simulink model "Universal_ELC_for_MicroHydoPlant"  (R2025a)
settings: Solver=ode45  StartTime=0.0  StopTime=2  RelTol=1e-3
undefined symbols (not defined in the file): R_user
libraries: spsCurrentMeasurementLib x13, spsSeriesRLCBranchLib x9, spsMosfetLib x7, spsVoltageMeasurementLib x5, spsUniversalBridgeLib x3, spsPower3phInstantaneousLib x3, spsControlledVoltageSourceLib x3, spsThreePhaseSeriesRLCBranchLib x2, slpidlib x2, spsTHDLib x2, spsRMSLib x1, spsGroundLib x1
settings Model: Creator=Niranjan  LastModifiedBy=SimuVerity Contributors
settings SolverCC: AlgebraicLoopSolver=TrustRegion
settings DataIOCC: SaveFormat=StructureWithTime  ReturnWorkspaceOutputs=off
settings OptimizationCC: LifeSpan=inf
settings DebuggingCC: UnconnectedInputMsg=warning  UnconnectedOutputMsg=warning  UnconnectedLineMsg=warning  SFExecutionAtInitializationDiag=none  ArithmeticOperatorsInVariantConditions=warning
settings HardwareCC: ProdBitPerSizeT=32.0  ProdBitPerPtrDiffT=32.0  ProdWordSize=32.0  ProdHWDeviceType=Specified
settings ModelReferenceCC: EnableRefExpFcnMdlSchedulingChecks=on
settings SFSimCC: SimUseLocalCustomCode=off  CustomCodeUndefinedFunction=UseInterfaceOnly
settings RTWCC: RTWUseLocalCustomCode=off  GPUComputeCapability=3.5
settings CodeAppCC: StateflowObjectComments=on
settings SimscapeCC: SimscapeNormalizeSystem=off

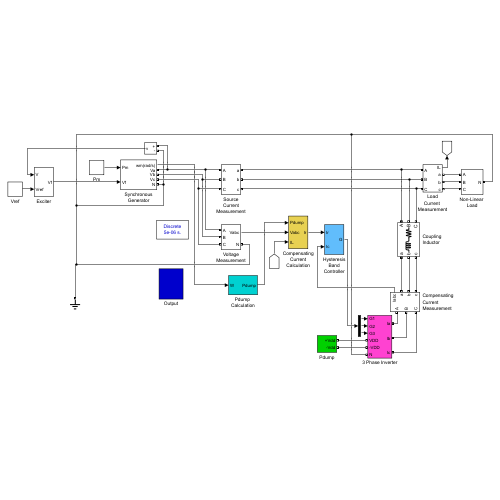
[thumbnail: Simulink's stored preview of the top-level diagram]
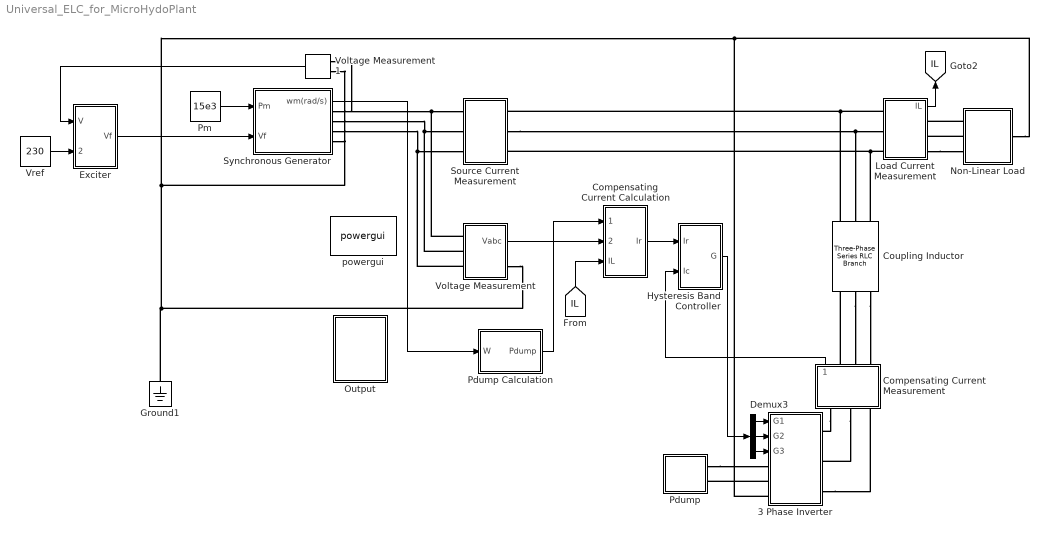
== system Universal_ELC_for_MicroHydoPlant ==
  3 Phase Inverter : Subsystem
  Compensating Current Calculation : Subsystem
  Compensating Current Measurement : Subsystem
  Coupling Inductor : spsThreePhaseSeriesRLCBranchLib/Three-Phase Series RLC Branch  LConnTagsString=A|B|C  RConnTagsString=A|B|C  BranchType=RL  Resistance=0.5  Inductance=0.015  Capacitance=1e-6  Measurements=None
  Demux3 : Demux  Outputs=3
  Exciter : Subsystem
  Ground1 : spsGroundLib/Ground  LConnTagsString=a
  Hysteresis Band Controller : Subsystem
  Load Current Measurement : Subsystem
  "Non-Linear Load " : Subsystem
  Output : Subsystem
  Pdump : Subsystem
  Pdump Calculation : Subsystem
  Pm : Constant  Value=15e3
  Source Current Measurement : Subsystem
  Synchronous Generator : Subsystem
  Voltage Measurement : Subsystem
  Voltage Measurement1 : spsVoltageMeasurementLib/Voltage Measurement  PhasorSimulation=off  OutputType=Complex  PSBequivalent=0
  Vref : Constant  Value=230
  powergui : spspowerguiLib/powergui  Priority=1  SimulationMode=Discrete  SampleTime=5e-6  frequency=60  Iterations=50  frequencyindice=0  Pbase=100e6  ErrMax=1e-4  UnitsV=kV  UnitsW=MW  buscounter=0  FunctionMessages=off  echomessages=off  EnableUseOfTLC=off  CurrentSourceSwitches=off  DisableSnubberDevices=off  DisableRonSwitches=off  DisableVfSwitches=off  DisplayEquations=off  AutomaticDiscreteSolvers=off  SolverType=Backward Euler  Interpol=off  ExternalGateDelay=off  methode=off  Ts=0  x0status=blocks  SPID=off  SwTol=0  HookPort=off  NonlinearTolerance=1e-4  nMaxIteration=100  ContinueOnMaxIteration=off  RestoreLinks=warning  ResistiveCurrentMeasurement=off  Frange=[0:2:500]  Ylog=off  Xlog=on  ShowGrid=off  save=off  variable=ZData  structure=0  ZoomFFT=off  StartTime=0.0  cycles=1  DisplayStyle=1  fundamental=60  FreqAxis=off  MaxFrequency=1000  frequencyindicesteady=1  RmsSteady=1  display=off
  tag scope: IL=global
  wires:
  Demux3/1 -> 3 Phase Inverter/1(G1)
  Demux3/2 -> 3 Phase Inverter/2(G2)
  Demux3/3 -> 3 Phase Inverter/3(G3)
  Hysteresis Band Controller/1(G) -> Demux3/1
  Compensating Current Measurement/1(Iabc) -> Hysteresis Band Controller/2(Ic)
  Compensating Current Calculation/1(Ir) -> Hysteresis Band Controller/1(Ir)
  Pdump Calculation/1(Pdump) -> Compensating Current Calculation/1(Pdump)
  Voltage Measurement/1(Vabc) -> Compensating Current Calculation/2(Vabc)
  Load Current Measurement/1(IL) -> [IL]
  [IL] -> Compensating Current Calculation/3(IL)
  Pm/1 -> Synchronous Generator/1(Pm)
  Synchronous Generator/1(wm(rad/s)) -> Pdump Calculation/1(W)
  Voltage Measurement1/1 -> Exciter/1(V)
  Vref/1 -> Exciter/2(Vref)
  Exciter/1(Vf) -> Synchronous Generator/2(Vf)
  connections:
  Compensating Current Measurement/LConn1 -- 3 Phase Inverter/RConn1
  Voltage Measurement/LConn1 -- Voltage Measurement1/LConn1 -- Synchronous Generator/RConn1 -- Source Current Measurement/LConn1
  3 Phase Inverter/RConn3 -- Compensating Current Measurement/LConn3
  Compensating Current Measurement/LConn2 -- 3 Phase Inverter/RConn2
  Compensating Current Measurement/RConn1 -- Coupling Inductor/RConn1
  Coupling Inductor/RConn2 -- Compensating Current Measurement/RConn2
  "Non-Linear Load "/LConn1 -- Load Current Measurement/RConn1
  Coupling Inductor/RConn3 -- Compensating Current Measurement/RConn3
  Load Current Measurement/RConn3 -- "Non-Linear Load "/LConn3
  Voltage Measurement/LConn2 -- Synchronous Generator/RConn2 -- Source Current Measurement/LConn2
  Pdump/RConn1 -- 3 Phase Inverter/LConn1
  3 Phase Inverter/LConn2 -- Pdump/RConn2
  Load Current Measurement/LConn1 -- Coupling Inductor/LConn1 -- Source Current Measurement/RConn1
  Load Current Measurement/LConn3 -- Coupling Inductor/LConn3 -- Source Current Measurement/RConn3
  Voltage Measurement/LConn3 -- Synchronous Generator/RConn3 -- Source Current Measurement/LConn3
  Voltage Measurement/RConn1 -- Ground1/LConn1 -- Voltage Measurement1/LConn2 -- Synchronous Generator/RConn4 -- "Non-Linear Load "/RConn1 -- 3 Phase Inverter/LConn3
  Source Current Measurement/RConn2 -- Coupling Inductor/LConn2 -- Load Current Measurement/LConn2
  "Non-Linear Load "/LConn2 -- Load Current Measurement/RConn2

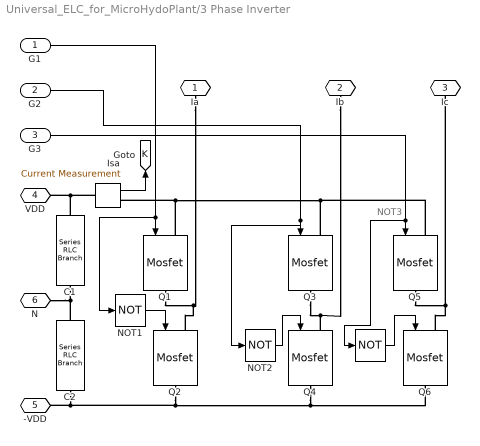
== system Universal_ELC_for_MicroHydoPlant/3 Phase Inverter ==
  note: NOT3
  G1 : Inport
  G2 : Inport  Port=2
  G3 : Inport  Port=3
  " " : Logic  Operator=NOT  AllPortsSameDT=off  OutDataTypeStr=boolean
  C1 : spsSeriesRLCBranchLib/Series RLC Branch  LConnTagsString=__new0  RConnTagsString=__new0  BranchType=C  Resistance=1  Inductance=1e-3  SetiL0=off  InitialCurrent=0  Capacitance=4700e-6  Setx0=on  InitialVoltage=500  Measurements=None
  C2 : spsSeriesRLCBranchLib/Series RLC Branch  LConnTagsString=__new0  RConnTagsString=__new0  BranchType=C  Resistance=1  Inductance=1e-3  SetiL0=off  InitialCurrent=0  Capacitance=4700e-6  Setx0=on  InitialVoltage=500  Measurements=None
  Isa : spsCurrentMeasurementLib/Current Measurement  PhasorSimulation=off  OutputType=Complex  PSBequivalent=0
  NOT1 : Logic  Operator=NOT  AllPortsSameDT=off  OutDataTypeStr=boolean
  NOT2 : Logic  Operator=NOT  AllPortsSameDT=off  OutDataTypeStr=boolean
  Q{1..6} (6 alike) : spsMosfetLib/Mosfet  Ron=0.01  Lon=0  Rd=0.01  Vfd=0  IC=0  Rs=1e10  Cs=inf  Measurements=off
  Ia : PMIOPort  Side=Right
  Ib : PMIOPort  Port=2  Side=Right
  Ic : PMIOPort  Port=3  Side=Right
  VDD : PMIOPort  Port=4  Side=Left
  -VDD : PMIOPort  Port=5  Side=Left
  N : PMIOPort  Port=6  Side=Left
  tag scope: K=global
  wires:
  NOT1/1 -> Q2/1
  NOT2/1 -> Q4/1
  " "/1 -> Q6/1
  G1/1 -> NOT1/1, Q1/1
  G2/1 -> Q3/1, NOT2/1
  G3/1 -> Q5/1, " "/1
  Isa/1 -> [K]
  connections:
  Q1/RConn1 -- Ia/RConn1 -- Q2/LConn1
  Isa/LConn1 -- VDD/RConn1 -- C1/LConn1
  Q3/RConn1 -- Ib/RConn1 -- Q4/LConn1
  Q2/RConn1 -- C2/RConn1 -- -VDD/RConn1 -- Q4/RConn1 -- Q6/RConn1
  Q6/LConn1 -- Ic/RConn1 -- Q5/RConn1
  Q1/LConn1 -- Isa/RConn1 -- Q5/LConn1 -- Q3/LConn1
  C2/LConn1 -- C1/RConn1 -- N/RConn1

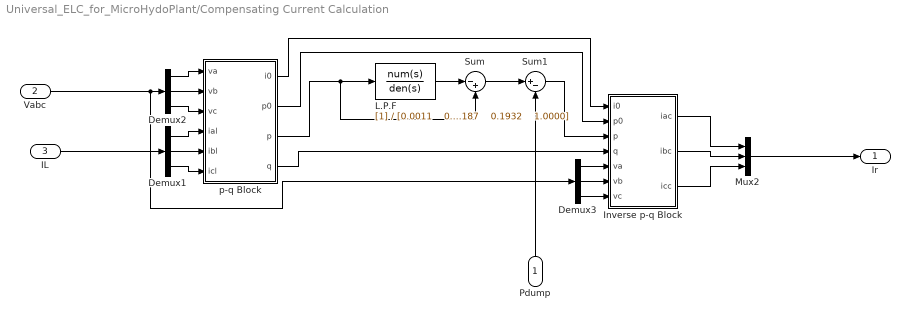
== system Universal_ELC_for_MicroHydoPlant/Compensating Current Calculation ==
  Pdump : Inport
  Vabc : Inport  Port=2
  IL : Inport  Port=3
  Demux1 : Demux  Outputs=3
  Demux2 : Demux  Outputs=3
  Demux3 : Demux  Outputs=3
  Inverse p-q Block : MATLAB Function  TreatAsAtomicUnit=on
  L.P.F : TransferFcn  Denominator="[0.0011    0.0187    0.1932    1.0000]"
  Mux2 : Mux  Inputs=3
  Sum : Sum  Inputs=|-+
  Sum1 : Sum  Inputs=|+-
  p-q Block : MATLAB Function  TreatAsAtomicUnit=on
  Ir : Outport
  wires:
  Inverse p-q Block/3(icc) -> Mux2/3
  IL/1 -> Demux1/1
  Demux1/2 -> p-q Block/5(ibl)
  Mux2/1 -> Ir/1
  Inverse p-q Block/1(iac) -> Mux2/1
  Demux1/1 -> p-q Block/4(ial)
  Inverse p-q Block/2(ibc) -> Mux2/2
  p-q Block/1(i0) -> Inverse p-q Block/1(i0)
  p-q Block/3(p) -> L.P.F/1, Sum/2
  Pdump/1 -> Sum1/2
  L.P.F/1 -> Sum/1
  Sum/1 -> Sum1/1
  Sum1/1 -> Inverse p-q Block/3(p)
  p-q Block/4(q) -> Inverse p-q Block/4(q)
  Demux1/3 -> p-q Block/6(icl)
  p-q Block/2(p0) -> Inverse p-q Block/2(p0)
  Demux2/3 -> p-q Block/3(vc)
  Demux2/2 -> p-q Block/2(vb)
  Demux2/1 -> p-q Block/1(va)
  Vabc/1 -> Demux3/1, Demux2/1
  Demux3/1 -> Inverse p-q Block/5(va)
  Demux3/2 -> Inverse p-q Block/6(vb)
  Demux3/3 -> Inverse p-q Block/7(vc)

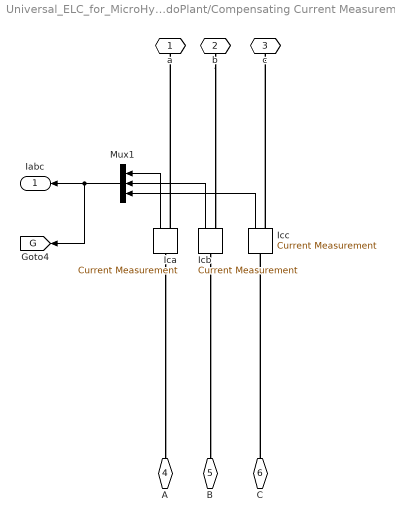
== system Universal_ELC_for_MicroHydoPlant/Compensating Current Measurement ==
  Ica : spsCurrentMeasurementLib/Current Measurement  PhasorSimulation=off  OutputType=Complex  PSBequivalent=0
  Icb : spsCurrentMeasurementLib/Current Measurement  PhasorSimulation=off  OutputType=Complex  PSBequivalent=0
  Icc : spsCurrentMeasurementLib/Current Measurement  PhasorSimulation=off  OutputType=Complex  PSBequivalent=0
  Mux1 : Mux  Inputs=3
  a : PMIOPort  Side=Right
  b : PMIOPort  Port=2  Side=Right
  c : PMIOPort  Port=3  Side=Right
  A : PMIOPort  Port=4  Side=Left
  B : PMIOPort  Port=5  Side=Left
  C : PMIOPort  Port=6  Side=Left
  Iabc : Outport
  tag scope: G=global
  wires:
  Mux1/1 -> [G], Iabc/1
  Ica/1 -> Mux1/1
  Icc/1 -> Mux1/3
  Icb/1 -> Mux1/2
  connections:
  b/RConn1 -- Icb/RConn1
  Ica/RConn1 -- a/RConn1
  Icc/RConn1 -- c/RConn1
  C/RConn1 -- Icc/LConn1
  Ica/LConn1 -- A/RConn1
  Icb/LConn1 -- B/RConn1

== system Universal_ELC_for_MicroHydoPlant/Exciter ==
  V : Inport
  Vref : Inport  Port=2
  PI Controller : slpidlib/PID Controller  Controller=PI  Form=Parallel  TimeDomain=Continuous-time  UseExternalTs=off  SampleTime=-1  IntegratorMethod=Forward Euler  FilterMethod=Forward Euler  ControllerParametersSource=internal  P=8  I=6  UseKiTs=off  D=0  UseExternalDerivativeSource=off  N=100  UseFilter=on  TunerSelectOption=Transfer Function Based (PID Tuner App)  InitialConditionSource=internal  InitialConditionForIntegrator=0  InitialConditionForFilter=0  DifferentiatorICPrevScaledInput=0  ExternalReset=none  TrackingMode=off  Kt=1  LimitOutput=off  SatLimitsSource=internal  UpperSaturationLimit=inf  LowerSaturationLimit=-inf  LinearizeAsGain=on  AntiWindupMode=none  Kb=1  LimitIntegrator=off  UpperIntegratorSaturationLimit=inf  LowerIntegratorSaturationLimit=-inf  POutMin=[]  POutMax=[]  IOutMin=[]  IOutMax=[]  DOutMin=[]  DOutMax=[]  NOutMin=[]  NOutMax=[]  SumOutMin=[]  SumOutMax=[]  SaturationOutMin=[]  SaturationOutMax=[]  PParamMin=[]  PParamMax=[]  IParamMin=[]  IParamMax=[]  DParamMin=[]  DParamMax=[]  NParamMin=[]  NParamMax=[]  KbParamMin=[]  KbParamMax=[]  KtParamMin=[]  KtParamMax=[]  KbOutMin=[]  KbOutMax=[]  KtOutMin=[]  KtOutMax=[]  IntegratorOutMin=[]  IntegratorOutMax=[]  FilterOutMin=[]  FilterOutMax=[]  SumI1OutMin=[]  SumI1OutMax=[]  SumI2OutMin=[]  SumI2OutMax=[]  SumI3OutMin=[]  SumI3OutMax=[]  SumI4OutMin=[]  SumI4OutMax=[]  SumDOutMin=[]  SumDOutMax=[]  DifferentiatorOutMin=[]  DifferentiatorOutMax=[]  FilterDiffOutCoefMin=[]  FilterDiffOutCoefMax=[]  ReciprocalOutMin=[]  ReciprocalOutMax=[]  SumDenOutMin=[]  SumDenOutMax=[]  SumNumOutMin=[]  SumNumOutMax=[]  DivideOutMin=[]  DivideOutMax=[]  UdiffTsProdOutMin=[]  UdiffTsProdOutMax=[]  NTsProdOutMin=[]  NTsProdOutMax=[]  UintegralTsProdOutMin=[]  UintegralTsProdOutMax=[]  UngainTsProdOutMin=[]  UngainTsProdOutMax=[]  ClampingZeroOutDataTypeStr=Inherit: Inherit via back propagation  ClampingZeroOutMin=[]  ClampingZeroOutMax=[]  FilterDenConstantOutDataTypeStr=Inherit: Inherit via back propagation  FilterDenConstantOutMin=[]  FilterDenConstantOutMax=[]  PCopyOutDataTypeStr=Inherit: Inherit via back propagation  PCopyOutMin=[]  PCopyOutMax=[]  NCopyOutDataTypeStr=Inherit: Inherit via back propagation  NCopyOutMin=[]  NCopyOutMax=[]  IntegratorContinuousStateAttributes=''  IntegratorStateMustResolveToSignalObject=off  IntegratorRTWStateStorageClass=Auto  FilterContinuousStateAttributes=''  FilterStateMustResolveToSignalObject=off  FilterRTWStateStorageClass=Auto  ParallelPVariant=InternalParameters  IdealPVariant=Disabled  IVariant=InternalParameters  DVariant=Disabled  IntegratorVariant=Continuous  SatVariant=Disabled  AWVariant=Passthrough  PCopyVariant=Disabled  TRVariant=Disabled  FdbkBlocksVariant=Forward  IdealPFdbkVariant=Disabled  SatFdbkVariant=Disabled  DerivativeFilterVariant=Disabled  NVariant=Disabled  NCopyVariant=Disabled_SignalSpec  FilterICVariant=Disabled  IntegratorICVariant=InternalICs  ExternalResetVariant=Disabled  TRSumVariant=Passthrough  SumFdbkVariant=Disabled  SumVariant=Sum_PI  TsampFilterVariant=InternalTs  TsampNgainVariant=Passthrough  TsampIntegralVariant=Disabled_SignalSpec  ExternalSaturationOutDataTypeStr=Inherit: Same as second input  DerivativeSourceVariant=Disabled  PreIntVariant=InternalPreInt
  RMS : spsRMSLib/RMS  TrueRMS=on  Freq=50  RMSInit=120  Ts=0
  Sum : Sum  Inputs=-+|
  Vf : Outport
  wires:
  V/1 -> RMS/1
  PI Controller/1 -> Vf/1
  Sum/1 -> PI Controller/1
  RMS/1 -> Sum/1
  Vref/1 -> Sum/2

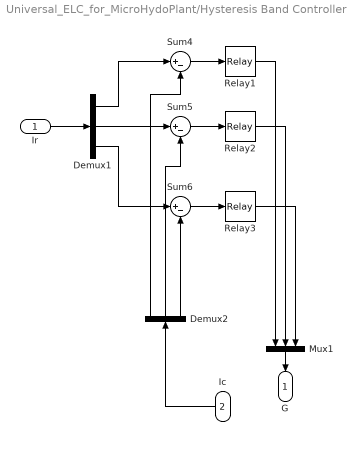
== system Universal_ELC_for_MicroHydoPlant/Hysteresis Band Controller ==
  Ir : Inport
  Ic : Inport  Port=2
  Demux1 : Demux  Outputs=3
  Demux2 : Demux  Outputs=3
  Mux1 : Mux  Inputs=3
  Relay1 : Relay  OnSwitchValue=0.1  OffSwitchValue=-0.2  ZeroCross=off
  Relay2 : Relay  OnSwitchValue=0.2  OffSwitchValue=-0.2  ZeroCross=off
  Relay3 : Relay  OnSwitchValue=0.2  OffSwitchValue=-0.2  ZeroCross=off
  Sum4 : Sum  Inputs=|+-
  Sum5 : Sum  Inputs=|+-
  Sum6 : Sum  Inputs=|+-
  G : Outport
  wires:
  Relay3/1 -> Mux1/3
  Relay1/1 -> Mux1/1
  Relay2/1 -> Mux1/2
  Demux2/2 -> Sum5/2
  Demux1/2 -> Sum5/1
  Sum6/1 -> Relay3/1
  Demux1/1 -> Sum4/1
  Demux1/3 -> Sum6/1
  Demux2/3 -> Sum6/2
  Sum5/1 -> Relay2/1
  Demux2/1 -> Sum4/2
  Sum4/1 -> Relay1/1
  Mux1/1 -> G/1
  Ir/1 -> Demux1/1
  Ic/1 -> Demux2/1

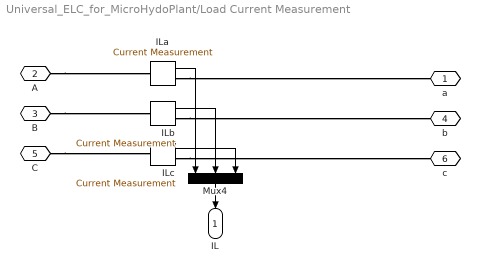
== system Universal_ELC_for_MicroHydoPlant/Load Current Measurement ==
  ILa : spsCurrentMeasurementLib/Current Measurement  PhasorSimulation=off  OutputType=Complex  PSBequivalent=0
  ILb : spsCurrentMeasurementLib/Current Measurement  PhasorSimulation=off  OutputType=Complex  PSBequivalent=0
  ILc : spsCurrentMeasurementLib/Current Measurement  PhasorSimulation=off  OutputType=Complex  PSBequivalent=0
  Mux4 : Mux  Inputs=3
  a : PMIOPort  Side=Right
  A : PMIOPort  Port=2  Side=Left
  B : PMIOPort  Port=3  Side=Left
  b : PMIOPort  Port=4  Side=Right
  C : PMIOPort  Port=5  Side=Left
  c : PMIOPort  Port=6  Side=Right
  IL : Outport
  wires:
  Mux4/1 -> IL/1
  ILa/1 -> Mux4/1
  ILc/1 -> Mux4/3
  ILb/1 -> Mux4/2
  connections:
  ILb/RConn1 -- b/RConn1
  ILa/RConn1 -- a/RConn1
  ILc/RConn1 -- c/RConn1
  A/RConn1 -- ILa/LConn1
  C/RConn1 -- ILc/LConn1
  B/RConn1 -- ILb/LConn1

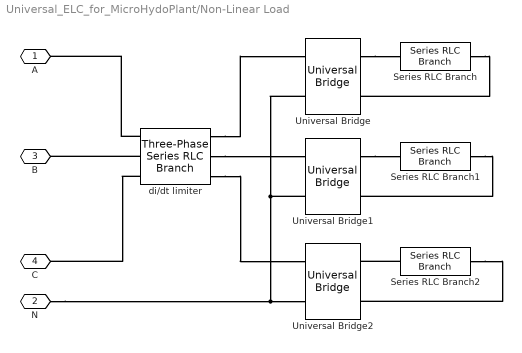
== system Universal_ELC_for_MicroHydoPlant/Non-Linear Load  ==
  Series RLC Branch : spsSeriesRLCBranchLib/Series RLC Branch  LConnTagsString=__new0  RConnTagsString=__new0  BranchType=RL  Resistance=R_user  Inductance=0.5  SetiL0=off  InitialCurrent=0  Capacitance=1e-6  Setx0=off  InitialVoltage=0  Measurements=None
  Series RLC Branch1 : spsSeriesRLCBranchLib/Series RLC Branch  LConnTagsString=__new0  RConnTagsString=__new0  BranchType=RL  Resistance=13  Inductance=0.9  SetiL0=off  InitialCurrent=0  Capacitance=1e-6  Setx0=off  InitialVoltage=0  Measurements=None
  Series RLC Branch2 : spsSeriesRLCBranchLib/Series RLC Branch  LConnTagsString=__new0  RConnTagsString=__new0  BranchType=RL  Resistance=20  Inductance=0.8  SetiL0=off  InitialCurrent=0  Capacitance=1e-6  Setx0=off  InitialVoltage=0  Measurements=None
  Universal Bridge : spsUniversalBridgeLib/Universal Bridge  Arms=2  SnubberResistance=1e10  SnubberCapacitance=1e3  Device=Diodes  Ron=1e-2  Lon=0.1  ForwardVoltages="[  0  0  ]"  ForwardVoltage=5  GTOparameters=[ 10e-6 , 20e-6 ]  IGBTparameters=[ 1e-6 , 2e-6 ]  Measurements=None  Measurements_2=None  converterType=Rectifier
  Universal Bridge1 : spsUniversalBridgeLib/Universal Bridge  Arms=2  SnubberResistance=1e10  SnubberCapacitance=1e3  Device=Diodes  Ron=1e-2  Lon=0.1  ForwardVoltages="[  0  0  ]"  ForwardVoltage=5  GTOparameters=[ 10e-6 , 20e-6 ]  IGBTparameters=[ 1e-6 , 2e-6 ]  Measurements=None  Measurements_2=None  converterType=Rectifier
  Universal Bridge2 : spsUniversalBridgeLib/Universal Bridge  Arms=2  SnubberResistance=1e10  SnubberCapacitance=1e3  Device=Diodes  Ron=1e-2  Lon=0.1  ForwardVoltages="[  0  0  ]"  ForwardVoltage=5  GTOparameters=[ 10e-6 , 20e-6 ]  IGBTparameters=[ 1e-6 , 2e-6 ]  Measurements=None  Measurements_2=None  converterType=Rectifier
  di/dt limiter : spsThreePhaseSeriesRLCBranchLib/Three-Phase Series RLC Branch  LConnTagsString=A|B|C  RConnTagsString=A|B|C  BranchType=L  Resistance=0.05  Inductance=10e-4  Capacitance=1e-6  Measurements=None
  A : PMIOPort  Side=Left
  N : PMIOPort  Port=2  Side=Right
  B : PMIOPort  Port=3  Side=Left
  C : PMIOPort  Port=4  Side=Left
  connections:
  Universal Bridge1/RConn1 -- Series RLC Branch1/LConn1
  Universal Bridge/RConn1 -- Series RLC Branch/LConn1
  Series RLC Branch2/LConn1 -- Universal Bridge2/RConn1
  Series RLC Branch2/RConn1 -- Universal Bridge2/RConn2
  Series RLC Branch1/RConn1 -- Universal Bridge1/RConn2
  Series RLC Branch/RConn1 -- Universal Bridge/RConn2
  Universal Bridge/LConn2 -- Universal Bridge1/LConn2 -- N/RConn1 -- Universal Bridge2/LConn2
  di/dt limiter/RConn1 -- A/RConn1
  di/dt limiter/RConn2 -- B/RConn1
  di/dt limiter/LConn2 -- Universal Bridge1/LConn1
  di/dt limiter/RConn3 -- C/RConn1
  di/dt limiter/LConn3 -- Universal Bridge2/LConn1
  di/dt limiter/LConn1 -- Universal Bridge/LConn1

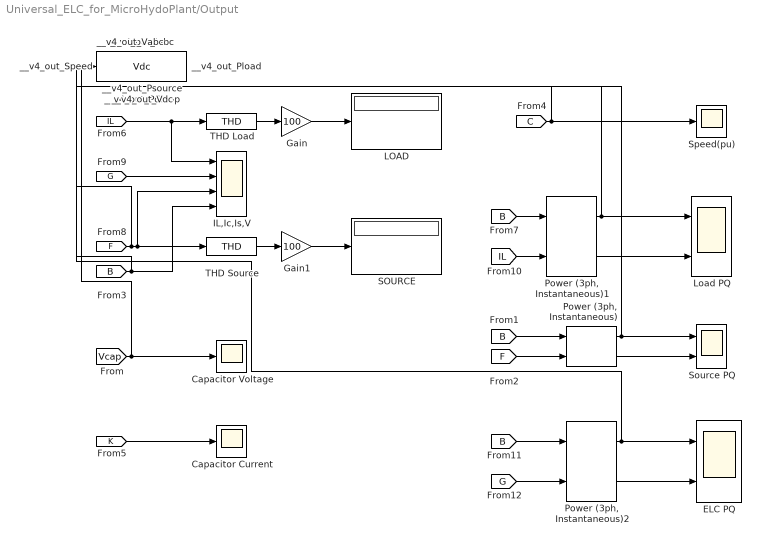
== system Universal_ELC_for_MicroHydoPlant/Output ==
  Capacitor Current : Scope
      settings: ActiveDisplayYMinimum=-52.5254  ActiveDisplayYMaximum=48.94509
  Capacitor Voltage : Scope
      settings: ActiveDisplayYMinimum=968.49867  ActiveDisplayYMaximum=1031.37394  DataLoggingSaveFormat=Array
  ELC PQ : Scope  NumInputPorts=2
      settings: ActiveDisplayYMinimum=-10122.15669  ActiveDisplayYMaximum=-3494.34994  DataLoggingVariableName=ScopeData2  DataLoggingSaveFormat=Array
  Gain : Gain  Gain=100
  Gain1 : Gain  Gain=100
  IL,Ic,Is,V : Scope  NumInputPorts=4
      settings: ActiveDisplayYMinimum=-24.30805  ActiveDisplayYMaximum=24.30926  DataLoggingMaxPoints=0.5e+5
  LOAD : Display
  Load PQ : Scope  NumInputPorts=2
      settings: ActiveDisplayYMinimum=-1303.81999  ActiveDisplayYMaximum=11734.37994  DataLoggingVariableName=ScopeData2
  "Power (3ph, Instantaneous)" : spsPower3phInstantaneousLib/Power (3ph, Instantaneous)
  "Power (3ph, Instantaneous)1" : spsPower3phInstantaneousLib/Power (3ph, Instantaneous)
  "Power (3ph, Instantaneous)2" : spsPower3phInstantaneousLib/Power (3ph, Instantaneous)
  SOURCE : Display
  Source PQ : Scope  NumInputPorts=2
      settings: ActiveDisplayYMinimum=-2171.90166  ActiveDisplayYMaximum=19150.12146
  Speed(pu) : Scope
      settings: ActiveDisplayYMinimum=0.99817  ActiveDisplayYMaximum=1.01245  DataLoggingVariableName=ScopeData3
  THD Load : spsTHDLib/THD  Freq=50  Ts=0
  THD Source : spsTHDLib/THD  Freq=50  Ts=0
  __v4_out_Iabc : ToWorkspace  VariableName=Iabc  SaveFormat=Timeseries  SampleTime=-1
  __v4_out_Pdump : ToWorkspace  VariableName=Pdump  SaveFormat=Timeseries  SampleTime=-1
  __v4_out_Pload : ToWorkspace  VariableName=Pload  SaveFormat=Timeseries  SampleTime=-1
  __v4_out_Psource : ToWorkspace  VariableName=Psource  SaveFormat=Timeseries  SampleTime=-1
  __v4_out_Speed : ToWorkspace  VariableName=Speed  SaveFormat=Timeseries  SampleTime=-1
  __v4_out_Vabc : ToWorkspace  VariableName=Vabc  SaveFormat=Timeseries  SampleTime=-1
  __v4_out_Vdc : ToWorkspace  VariableName=Vdc  SaveFormat=Timeseries  SampleTime=-1
  wires:
  THD Source/1 -> Gain1/1
  THD Load/1 -> Gain/1
  [C] -> Speed(pu)/1, __v4_out_Speed/1
  [F] -> IL,Ic,Is,V/3, THD Source/1, __v4_out_Iabc/1
  [IL] -> IL,Ic,Is,V/1, THD Load/1
  Gain/1 -> LOAD/1
  Gain1/1 -> SOURCE/1
  [B] -> IL,Ic,Is,V/4, __v4_out_Vabc/1
  [G] -> IL,Ic,Is,V/2
  [K] -> Capacitor Current/1
  [B] -> "Power (3ph, Instantaneous)"/1
  [F] -> "Power (3ph, Instantaneous)"/2
  "Power (3ph, Instantaneous)"/2 -> Source PQ/2
  [B] -> "Power (3ph, Instantaneous)1"/1
  [IL] -> "Power (3ph, Instantaneous)1"/2
  "Power (3ph, Instantaneous)1"/1 -> Load PQ/1, __v4_out_Pload/1
  "Power (3ph, Instantaneous)1"/2 -> Load PQ/2
  "Power (3ph, Instantaneous)"/1 -> Source PQ/1, __v4_out_Psource/1
  [Vcap] -> Capacitor Voltage/1, __v4_out_Vdc/1
  [B] -> "Power (3ph, Instantaneous)2"/1
  [G] -> "Power (3ph, Instantaneous)2"/2
  "Power (3ph, Instantaneous)2"/1 -> ELC PQ/1, __v4_out_Pdump/1
  "Power (3ph, Instantaneous)2"/2 -> ELC PQ/2

== system Universal_ELC_for_MicroHydoPlant/Pdump ==
  Constant : Constant  Value=1000
  Rdump : spsSeriesRLCBranchLib/Series RLC Branch  LConnTagsString=__new0  RConnTagsString=__new0  BranchType=R  Resistance=60  Inductance=0.0455  SetiL0=off  InitialCurrent=0  Capacitance=1e-6  Setx0=off  InitialVoltage=0  Measurements=None
  Relay : Relay  OnSwitchValue=25  OffSwitchValue=-25
  S : spsMosfetLib/Mosfet  Ron=0.1  Lon=0  Rd=0.01  Vfd=0  IC=0  Rs=1e5  Cs=inf  Measurements=off
  Sum : Sum  Inputs=|+-
  Vcap : spsVoltageMeasurementLib/Voltage Measurement  PhasorSimulation=off  OutputType=Complex  PSBequivalent=0
  +Vdd : PMIOPort  Side=Right
  -Vdd : PMIOPort  Port=2  Side=Right
  tag scope: Vcap=global
  wires:
  Vcap/1 -> Sum/1, [Vcap]
  Constant/1 -> Sum/2
  Sum/1 -> Relay/1
  Relay/1 -> S/1
  connections:
  -Vdd/RConn1 -- Vcap/LConn2 -- S/RConn1
  Vcap/LConn1 -- Rdump/LConn1 -- +Vdd/RConn1
  S/LConn1 -- Rdump/RConn1

== system Universal_ELC_for_MicroHydoPlant/Pdump Calculation ==
  W : Inport
  PI Controller : slpidlib/PID Controller  Controller=PI  Form=Parallel  TimeDomain=Discrete-time  UseExternalTs=off  SampleTime=0.0001  IntegratorMethod=Forward Euler  FilterMethod=Forward Euler  ControllerParametersSource=internal  P=8000  I=15000  UseKiTs=off  D=0  UseExternalDerivativeSource=off  N=100  UseFilter=on  TunerSelectOption=Transfer Function Based (PID Tuner App)  ZeroCross=off  InitialConditionSource=internal  InitialConditionForIntegrator=0  InitialConditionForFilter=0  DifferentiatorICPrevScaledInput=0  ExternalReset=none  TrackingMode=off  Kt=1  LimitOutput=off  SatLimitsSource=internal  UpperSaturationLimit=inf  LowerSaturationLimit=-inf  LinearizeAsGain=off  AntiWindupMode=none  Kb=1  LimitIntegrator=off  UpperIntegratorSaturationLimit=inf  LowerIntegratorSaturationLimit=-inf  POutMin=[]  POutMax=[]  IOutMin=[]  IOutMax=[]  DOutMin=[]  DOutMax=[]  NOutMin=[]  NOutMax=[]  SumOutMin=[]  SumOutMax=[]  SaturationOutMin=[]  SaturationOutMax=[]  PParamMin=[]  PParamMax=[]  IParamMin=[]  IParamMax=[]  DParamMin=[]  DParamMax=[]  NParamMin=[]  NParamMax=[]  KbParamMin=[]  KbParamMax=[]  KtParamMin=[]  KtParamMax=[]  KbOutMin=[]  KbOutMax=[]  KtOutMin=[]  KtOutMax=[]  IntegratorOutMin=[]  IntegratorOutMax=[]  FilterOutMin=[]  FilterOutMax=[]  SumI1OutMin=[]  SumI1OutMax=[]  SumI2OutMin=[]  SumI2OutMax=[]  SumI3OutMin=[]  SumI3OutMax=[]  SumI4OutMin=[]  SumI4OutMax=[]  SumDOutMin=[]  SumDOutMax=[]  DifferentiatorOutMin=[]  DifferentiatorOutMax=[]  FilterDiffOutCoefMin=[]  FilterDiffOutCoefMax=[]  ReciprocalOutMin=[]  ReciprocalOutMax=[]  SumDenOutMin=[]  SumDenOutMax=[]  SumNumOutMin=[]  SumNumOutMax=[]  DivideOutMin=[]  DivideOutMax=[]  UdiffTsProdOutMin=[]  UdiffTsProdOutMax=[]  NTsProdOutMin=[]  NTsProdOutMax=[]  UintegralTsProdOutMin=[]  UintegralTsProdOutMax=[]  UngainTsProdOutMin=[]  UngainTsProdOutMax=[]  ClampingZeroOutDataTypeStr=Inherit: Inherit via back propagation  ClampingZeroOutMin=[]  ClampingZeroOutMax=[]  FilterDenConstantOutDataTypeStr=Inherit: Inherit via back propagation  FilterDenConstantOutMin=[]  FilterDenConstantOutMax=[]  PCopyOutDataTypeStr=Inherit: Inherit via back propagation  PCopyOutMin=[]  PCopyOutMax=[]  NCopyOutDataTypeStr=Inherit: Inherit via back propagation  NCopyOutMin=[]  NCopyOutMax=[]  IntegratorContinuousStateAttributes=''  IntegratorStateMustResolveToSignalObject=off  IntegratorRTWStateStorageClass=Auto  FilterContinuousStateAttributes=''  FilterStateMustResolveToSignalObject=off  FilterRTWStateStorageClass=Auto  ParallelPVariant=InternalParameters  IdealPVariant=Disabled  IVariant=InternalParameters  DVariant=Disabled  IntegratorVariant=Discrete  SatVariant=Disabled  AWVariant=Passthrough  PCopyVariant=Disabled  TRVariant=Disabled  FdbkBlocksVariant=Forward  IdealPFdbkVariant=Disabled  SatFdbkVariant=Disabled  DerivativeFilterVariant=Disabled  NVariant=Disabled  NCopyVariant=Disabled_SignalSpec  FilterICVariant=Disabled  IntegratorICVariant=InternalICs  ExternalResetVariant=Disabled  TRSumVariant=Passthrough  SumFdbkVariant=Disabled  SumVariant=Sum_PI  TsampFilterVariant=InternalTs  TsampNgainVariant=Passthrough  TsampIntegralVariant=Disabled_SignalSpec  ExternalSaturationOutDataTypeStr=Inherit: Same as second input  DerivativeSourceVariant=Disabled  PreIntVariant=InternalPreInt
  Sum3 : Sum  Inputs=|-+
  Wref : Constant  Value=157
  w(p.u) : Gain  Gain=1/157
  Pdump : Outport
  tag scope: C=global
  wires:
  PI Controller/1 -> Pdump/1
  Wref/1 -> Sum3/1
  Sum3/1 -> PI Controller/1
  W/1 -> w(p.u)/1, Sum3/2
  w(p.u)/1 -> [C]

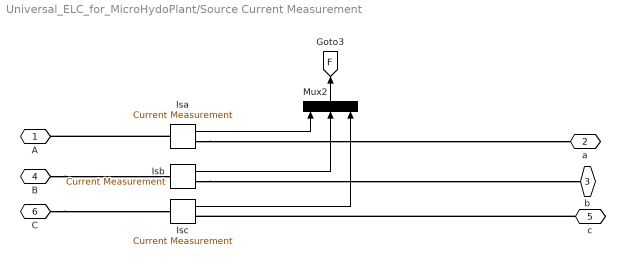
== system Universal_ELC_for_MicroHydoPlant/Source Current Measurement ==
  Isa : spsCurrentMeasurementLib/Current Measurement  PhasorSimulation=off  OutputType=Complex  PSBequivalent=0
  Isb : spsCurrentMeasurementLib/Current Measurement  PhasorSimulation=off  OutputType=Complex  PSBequivalent=0
  Isc : spsCurrentMeasurementLib/Current Measurement  PhasorSimulation=off  OutputType=Complex  PSBequivalent=0
  Mux2 : Mux  Inputs=3
  A : PMIOPort  Side=Left
  a : PMIOPort  Port=2  Side=Right
  b : PMIOPort  Port=3  Side=Right
  B : PMIOPort  Port=4  Side=Left
  c : PMIOPort  Port=5  Side=Right
  C : PMIOPort  Port=6  Side=Left
  tag scope: F=global
  wires:
  Isc/1 -> Mux2/3
  Isb/1 -> Mux2/2
  Isa/1 -> Mux2/1
  Mux2/1 -> [F]
  connections:
  Isa/RConn1 -- a/RConn1
  B/RConn1 -- Isb/LConn1
  Isb/RConn1 -- b/RConn1
  c/RConn1 -- Isc/RConn1
  C/RConn1 -- Isc/LConn1
  Isa/LConn1 -- A/RConn1

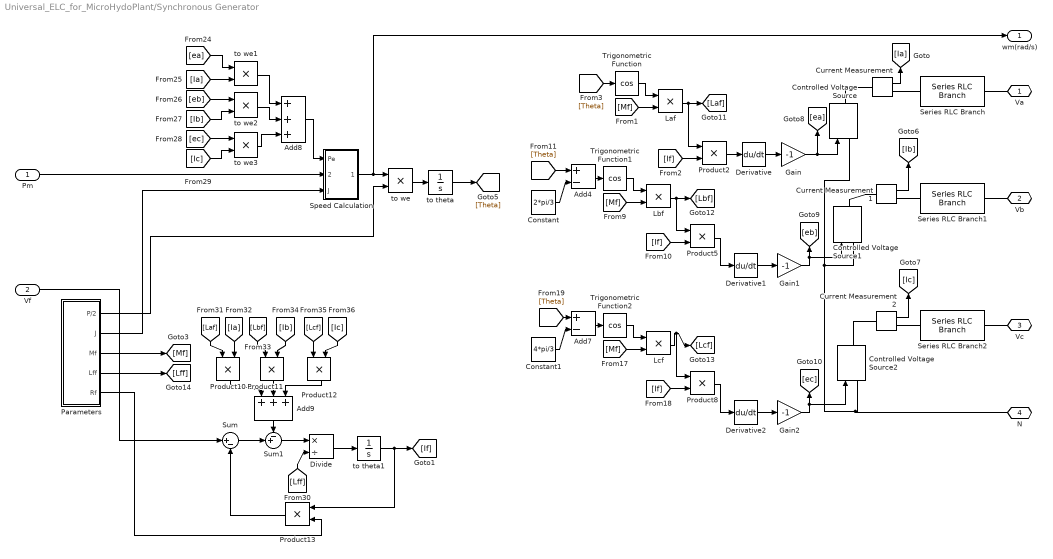
== system Universal_ELC_for_MicroHydoPlant/Synchronous Generator ==
  Pm : Inport
  Vf : Inport  Port=2
  Add4 : Sum  Inputs=+-
  Add7 : Sum  Inputs=+-
  Add8 : Sum  Inputs=+++
  Add9 : Sum  Inputs=+++
  Constant : Constant  Value=2*pi/3
  Constant1 : Constant  Value=4*pi/3
  Controlled Voltage Source : spsControlledVoltageSourceLib/Controlled Voltage Source  Initialize=on  Source_Type=AC  Amplitude=0  Phase=0  Frequency=0  Measurements=None
  Controlled Voltage Source1 : spsControlledVoltageSourceLib/Controlled Voltage Source  Initialize=on  Source_Type=AC  Amplitude=0  Phase=0  Frequency=0  Measurements=None
  Controlled Voltage Source2 : spsControlledVoltageSourceLib/Controlled Voltage Source  Initialize=on  Source_Type=AC  Amplitude=0  Phase=0  Frequency=0  Measurements=None
  Current Measurement : spsCurrentMeasurementLib/Current Measurement  PhasorSimulation=off  OutputType=Complex  PSBequivalent=0
  Current Measurement1 : spsCurrentMeasurementLib/Current Measurement  PhasorSimulation=off  OutputType=Complex  PSBequivalent=0
  Current Measurement2 : spsCurrentMeasurementLib/Current Measurement  PhasorSimulation=off  OutputType=Complex  PSBequivalent=0
  Derivative : Derivative
  Derivative1 : Derivative
  Derivative2 : Derivative
  Divide : Product  Inputs=*/
  Gain : Gain  Gain=-1
  Gain1 : Gain  Gain=-1
  Gain2 : Gain  Gain=-1
  Laf : Product
  Lbf : Product
  Lcf : Product
  Parameters : Subsystem
  Product{2,5,8,10..13} (7 alike) : Product
  Series RLC Branch : spsSeriesRLCBranchLib/Series RLC Branch  LConnTagsString=__new0  RConnTagsString=__new0  BranchType=RL  Resistance=0.01  Inductance=3e-4  SetiL0=off  InitialCurrent=0  Capacitance=1e-6  Setx0=off  InitialVoltage=0  Measurements=None
  Series RLC Branch1 : spsSeriesRLCBranchLib/Series RLC Branch  LConnTagsString=__new0  RConnTagsString=__new0  BranchType=RL  Resistance=0.01  Inductance=3e-4  SetiL0=off  InitialCurrent=0  Capacitance=1e-6  Setx0=off  InitialVoltage=0  Measurements=None
  Series RLC Branch2 : spsSeriesRLCBranchLib/Series RLC Branch  LConnTagsString=__new0  RConnTagsString=__new0  BranchType=RL  Resistance=0.01  Inductance=3e-4  SetiL0=off  InitialCurrent=0  Capacitance=1e-6  Setx0=off  InitialVoltage=0  Measurements=None
  Speed Calculation : Subsystem
  Sum : Sum  Inputs=|+-
  Sum1 : Sum  Inputs=-+|
  Trigonometric Function : Trigonometry  Operator=cos
  Trigonometric Function1 : Trigonometry  Operator=cos
  Trigonometric Function2 : Trigonometry  Operator=cos
  to theta : Integrator
  to theta1 : Integrator
  to we{,1..3} (4 alike) : Product
  Va : PMIOPort  Side=Right
  Vb : PMIOPort  Port=2  Side=Right
  Vc : PMIOPort  Port=3  Side=Right
  N : PMIOPort  Port=4  Side=Right
  wm(rad/s) : Outport
  wires:
  [ec] -> to we3/1
  Derivative/1 -> Gain/1
  Speed Calculation/1(wm) -> wm(rad/s)/1, to we/1
  Pm/1 -> Speed Calculation/2(Pm)
  Add4/1 -> Trigonometric Function1/1
  Lbf/1 -> [Lbf], Product5/1
  [If] -> Product5/2
  [Mf] -> Lbf/2
  Trigonometric Function1/1 -> Lbf/1
  Product5/1 -> Derivative1/1
  Current Measurement/1 -> [Ia]
  [Mf] -> Laf/2
  Add8/1 -> Speed Calculation/1(Pe)
  [Ib] -> to we2/2
  to we3/1 -> Add8/3
  [eb] -> to we2/1
  Laf/1 -> [Laf], Product2/1
  Add7/1 -> Trigonometric Function2/1
  Current Measurement2/1 -> [Ic]
  [Theta] -> Add4/1
  to we2/1 -> Add8/2
  Vf/1 -> Sum/1
  to we/1 -> to theta/1
  [Theta] -> Add7/1
  Constant/1 -> Add4/2
  Trigonometric Function/1 -> Laf/1
  Current Measurement1/1 -> [Ib]
  to theta/1 -> [Theta]
  [If] -> Product2/2
  Constant1/1 -> Add7/2
  [Mf] -> Lcf/2
  Trigonometric Function2/1 -> Lcf/1
  [If] -> Product8/2
  Product8/1 -> Derivative2/1
  [ea] -> to we1/1
  Lcf/1 -> [Lcf], Product8/1
  Product2/1 -> Derivative/1
  [Theta] -> Trigonometric Function/1
  Derivative1/1 -> Gain1/1
  [Ic] -> to we3/2
  [Ia] -> to we1/2
  to we1/1 -> Add8/1
  Sum/1 -> Sum1/2
  Product11/1 -> Add9/2
  Product10/1 -> Add9/1
  Product12/1 -> Add9/3
  Add9/1 -> Sum1/1
  Sum1/1 -> Divide/1
  [Lff] -> Divide/2
  Divide/1 -> to theta1/1
  to theta1/1 -> [If], Product13/1
  Product13/1 -> Sum/2
  [Laf] -> Product10/1
  [Ia] -> Product10/2
  [Lbf] -> Product11/1
  [Ib] -> Product11/2
  [Lcf] -> Product12/1
  [Ic] -> Product12/2
  Parameters/1(P/2) -> to we/2
  Parameters/2(J) -> Speed Calculation/3(J)
  Parameters/3(Mf) -> [Mf]
  Parameters/4(Lff) -> [Lff]
  Parameters/5(Rf) -> Product13/2
  Gain/1 -> [ea], Controlled Voltage Source/1
  Gain1/1 -> Controlled Voltage Source1/1, [eb]
  Derivative2/1 -> Gain2/1
  Gain2/1 -> Controlled Voltage Source2/1, [ec]
  connections:
  Current Measurement/RConn1 -- Series RLC Branch/LConn1
  Current Measurement1/LConn1 -- Controlled Voltage Source1/RConn1
  N/RConn1 -- Controlled Voltage Source2/LConn1 -- Controlled Voltage Source/LConn1 -- Controlled Voltage Source1/LConn1
  Series RLC Branch1/RConn1 -- Vb/RConn1
  Series RLC Branch2/RConn1 -- Vc/RConn1
  Series RLC Branch/RConn1 -- Va/RConn1
  Current Measurement/LConn1 -- Controlled Voltage Source/RConn1
  Series RLC Branch1/LConn1 -- Current Measurement1/RConn1
  Series RLC Branch2/LConn1 -- Current Measurement2/RConn1
  Current Measurement2/LConn1 -- Controlled Voltage Source2/RConn1

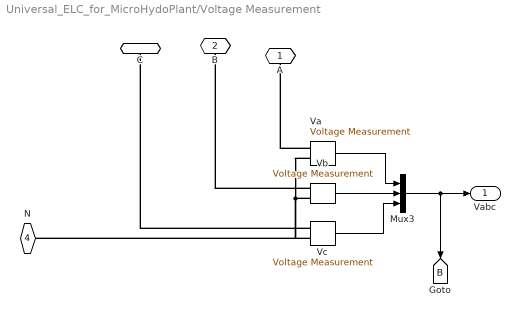
== system Universal_ELC_for_MicroHydoPlant/Voltage Measurement ==
  Mux3 : Mux  Inputs=3
  Va : spsVoltageMeasurementLib/Voltage Measurement  PhasorSimulation=off  OutputType=Complex  PSBequivalent=0
  Vb : spsVoltageMeasurementLib/Voltage Measurement  PhasorSimulation=off  OutputType=Complex  PSBequivalent=0
  Vc : spsVoltageMeasurementLib/Voltage Measurement  PhasorSimulation=off  OutputType=Complex  PSBequivalent=0
  A : PMIOPort  Side=Left
  B : PMIOPort  Port=2  Side=Left
  C : PMIOPort  Port=3  Side=Left
  N : PMIOPort  Port=4  Side=Right
  Vabc : Outport
  tag scope: B=global
  wires:
  Mux3/1 -> [B], Vabc/1
  Vc/1 -> Mux3/3
  Vb/1 -> Mux3/2
  Va/1 -> Mux3/1
  connections:
  Vc/LConn1 -- C/RConn1
  Vb/LConn1 -- B/RConn1
  Va/LConn1 -- A/RConn1
  Va/LConn2 -- Vc/LConn2 -- N/RConn1 -- Vb/LConn2

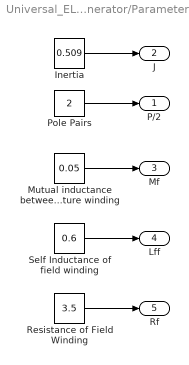
== system Universal_ELC_for_MicroHydoPlant/Synchronous Generator/Parameters ==
  Inertia : Constant  Value=0.509
  Mutual inductance between field and armature winding : Constant  Value=0.05
  Pole Pairs : Constant  Value=2
  Resistance of Field Winding : Constant  Value=3.5
  Self Inductance of field winding : Constant  Value=0.6
  P/2 : Outport
  J : Outport  Port=2
  Mf : Outport  Port=3
  Lff : Outport  Port=4
  Rf : Outport  Port=5
  wires:
  Inertia/1 -> J/1
  Mutual inductance between field and armature winding/1 -> Mf/1
  Self Inductance of field winding/1 -> Lff/1
  Pole Pairs/1 -> P/2/1
  Resistance of Field Winding/1 -> Rf/1

== system Universal_ELC_for_MicroHydoPlant/Synchronous Generator/Speed Calculation ==
  Pe : Inport
  Pm : Inport  Port=2
  J : Inport  Port=3
  Divide : Product  Inputs=*/
  Divide1 : Product  Inputs=*/
  Integrator : Integrator  InitialCondition=157
  Sum : Sum  Inputs=-+|
  wm : Outport
  wires:
  Sum/1 -> Divide/1
  Integrator/1 -> wm/1, Divide1/2
  J/1 -> Divide/2
  Pm/1 -> Sum/2
  Pe/1 -> Sum/1
  Divide/1 -> Divide1/1
  Divide1/1 -> Integrator/1

== matlab function Universal_ELC_for_MicroHydoPlant/Compensating Current Calculation/Inverse p-q Block ==
  data: i0 input; p0 input; p input; iac output; q input; va input; vb input; vc input; ibc output; icc output
function [iac,ibc,icc]= fcn(i0,p0,p,q,va,vb,vc)
%#codegen
v_zero=(va+vb+vc)/sqrt(3);
v_alpha=(va-vb/2-vc/2)*sqrt(2/3);
v_beta=(vb-vc)/sqrt(2);
i_zero=i0;
i_alpha=(v_alpha.*p+v_beta.*q)/(v_alpha.^2+v_beta.^2);
i_beta=(v_beta.*p-v_alpha.*q)/(v_alpha.^2+v_beta.^2);
iac=sqrt(2/3)*(i_zero/sqrt(2)+i_alpha);
ibc=sqrt(2/3)*(i_zero./sqrt(2)-i_alpha/2+sqrt(3)*i_beta/2);
icc=sqrt(2/3)*(i_zero./sqrt(2)-i_alpha/2-i_beta*sqrt(3)/2);

== matlab function Universal_ELC_for_MicroHydoPlant/Compensating Current Calculation/p-q Block ==
  data: i0 output; p0 output; va input; p output; vb input; vc input; ial input; ibl input; icl input; q output
function [i0,p0,p,q]= fcn(va,vb,vc,ial,ibl,icl)
%#codegen
v_zero=(va+vb+vc)/sqrt(3);
v_alpha=(va-vb/2-vc/2)*sqrt(2/3);
v_beta=(vb-vc)/sqrt(2);
il_zero=(ial+ibl+icl)/sqrt(3);
il_alpha=(ial-ibl/2-icl/2)*sqrt(2/3);
il_beta=(ibl-icl)/sqrt(2);
i0=il_zero;
p0=v_zero.*il_zero;
p=v_alpha.*il_alpha+v_beta.*il_beta;
q=v_beta.*il_alpha-v_alpha.*il_beta;
